simulink model "sf_atomic_sensor_pair"  (R2025b)
settings: Solver=FixedStepDiscrete  StartTime=0.0  StopTime=Inf  FixedStep=1  RelTol=1e-3  EnableMultiTasking=on
libraries: simulink x2, sf_atomic_sensor_lib x2
settings Model: Creator=The MathWorks, Inc.  LastModifiedBy=The MathWorks, Inc.
settings SolverCC: AlgebraicLoopSolver=TrustRegion
settings DataIOCC: LimitDataPoints=on  SaveFormat=Array  ReturnWorkspaceOutputs=off
settings OptimizationCC: ReuseModelBlockBuffer=off  ExpressionDepthLimit=2147483647.0  LifeSpan=inf
settings DebuggingCC: UnderspecifiedInitializationDetection=Classic  MergeDetectMultiDrivingBlocksExec=none  SolverPrmCheckMsg=warning  FcnCallInpInsideContextMsg=warning  UnconnectedInputMsg=warning  UnconnectedOutputMsg=warning  UnconnectedLineMsg=warning  StateNameClashWarn=warning  SFUnexpectedBacktrackingDiag=warning  SFNoUnconditionalDefaultTransitionDiag=warning  SFExecutionAtInitializationDiag=none  ArithmeticOperatorsInVariantConditions=warning
settings HardwareCC: ProdBitPerPointer=32.0  ProdBitPerSizeT=32.0  ProdBitPerPtrDiffT=32.0  ProdLargestAtomicFloat=None  ProdIntDivRoundTo=Undefined  ProdEndianess=Unspecified  ProdWordSize=32.0  ProdHWDeviceType=32-bit Generic
settings ModelReferenceCC: EnableRefExpFcnMdlSchedulingChecks=on  PropagateSignalLabelsOutOfModel=off
settings SFSimCC: SimUseLocalCustomCode=off  SimParseCustomCode=off  CustomCodeUndefinedFunction=UseInterfaceOnly
settings RTWCC: RTWUseLocalCustomCode=off  GPUComputeCapability=3.5
settings CodeAppCC: StateflowObjectComments=on
settings GRTTargetCC: TargetLangStandard=C89/C90 (ANSI)  CombineOutputUpdateFcns=off  GRTInterface=on
settings ConfigComp: CovMetricSettings=dw  CovSaveCumulativeToWorkspaceVar=on  CovSaveSingleToWorkspaceVar=on  CovExternalEMLEnable=off  CovSFcnEnable=off

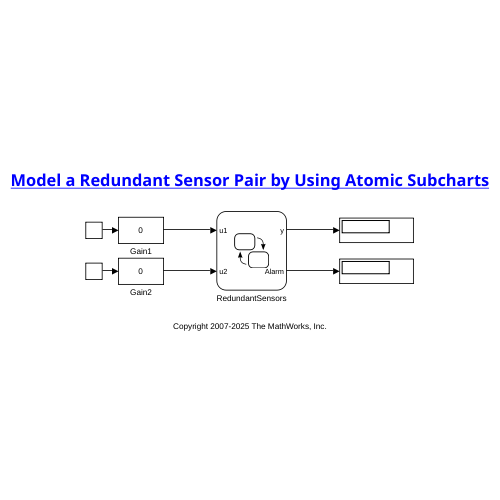
[thumbnail: Simulink's stored preview of the top-level diagram]
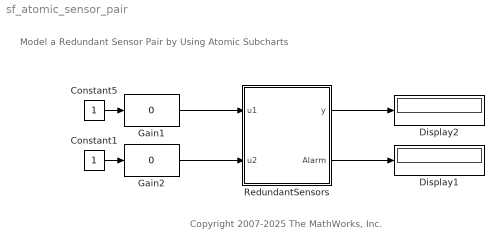
== system sf_atomic_sensor_pair ==
  note: Copyright 2007-2025 The MathWorks, Inc.
  note: Model a Redundant Sensor Pair by Using Atomic Subcharts
  Constant1 : Constant
  Constant5 : Constant
  Display1 : Display
  Display2 : Display
  Gain1 : simulink/Math Operations/Slider Gain  gain=0  low=-150  high=150
  Gain2 : simulink/Math Operations/Slider Gain  gain=0  low=-150  high=150
  RedundantSensors : Stateflow chart  TreatAsAtomicUnit=on
  wires:
  Constant5/1 -> Gain1/1
  Gain1/1 -> RedundantSensors/1(u1)
  Constant1/1 -> Gain2/1
  Gain2/1 -> RedundantSensors/2(u2)
  RedundantSensors/1(y) -> Display2/1
  RedundantSensors/2(" Alarm") -> Display1/1

== stateflow chart sf_atomic_sensor_pair/RedundantSensors ==
  state Sensor1
  state Sensor2
  state Alarm
    en, du: y = 0;
  (default) -> Sensor1
  Sensor1 -> Sensor2 : [Sensor1.inFailed()]
  Sensor2 -> Alarm : [Sensor2.inFailed()]
  data: u1 input; u2 input; y output double; Alarm output boolean
